simulink model "Exercise_1_2_model"  (R2025b)
settings: Solver=VariableStepAuto  StartTime=0.0  StopTime=0.30  RelTol=1e-3
undefined symbols (not defined in the file): L, R, R_V
settings Model: Creator=atharvaedake  LastModifiedBy=atharvaedake

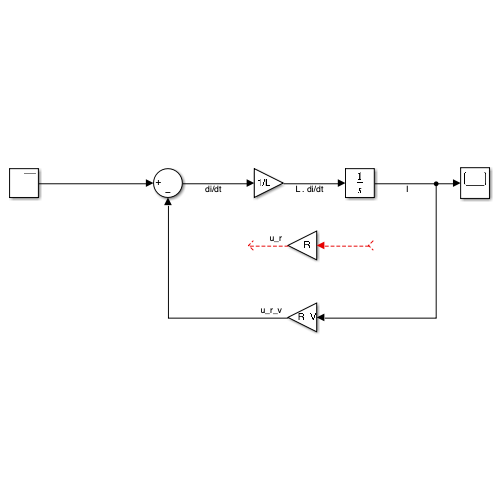
[thumbnail: Simulink's stored preview of the top-level diagram]
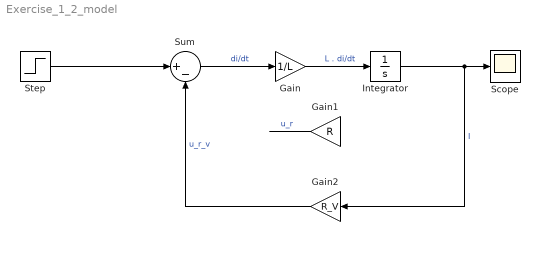
== system Exercise_1_2_model ==
  Gain : Gain  Gain=1/L
  Gain1 : Gain  Gain=R
  Gain2 : Gain  Gain=R_V
  Integrator : Integrator
  Scope : Scope
      settings: ActiveDisplayYMinimum=-2.6086880723680235  ActiveDisplayYMaximum=3.8808844205474466
  Step : Step  Time=0.1  After=10  SampleTime=0
  Sum : Sum  Inputs=|+-
  wires:
  Step/1 -> Sum/1
  Sum/1 -> Gain/1  "di/dt"
  Gain/1 -> Integrator/1  "L . di/dt"
  Integrator/1 -> Gain2/1, Scope/1  "I"
  Gain2/1 -> Sum/2  "u_r_v"
  Gain1/1 -> ?  "u_r"
  ? -> Gain1/1
